simulink model "gantry_2025a"  (R2025a)
settings: Solver=ode45  StartTime=0.0  StopTime=t(end)  RelTol=1e-4  AbsTol=1e-8
undefined symbols (not defined in the file): cb1, cb2, cc1, cc2, ccy, cg1, cg2, cy, d, Jb, Jh, kb1, kb2, Lb, Lh, m1, m2, mb, mh, P, ts, X, Y, Z
libraries: sm_lib x14, nesl_utility x10, cstblocks x3
settings Model: Creator=cocuser  LastModifiedBy=cocuser
settings DataIOCC: ReturnWorkspaceOutputs=off

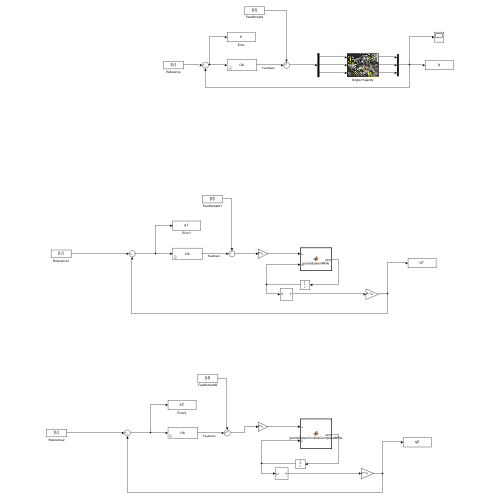
[thumbnail: Simulink's stored preview of the top-level diagram]
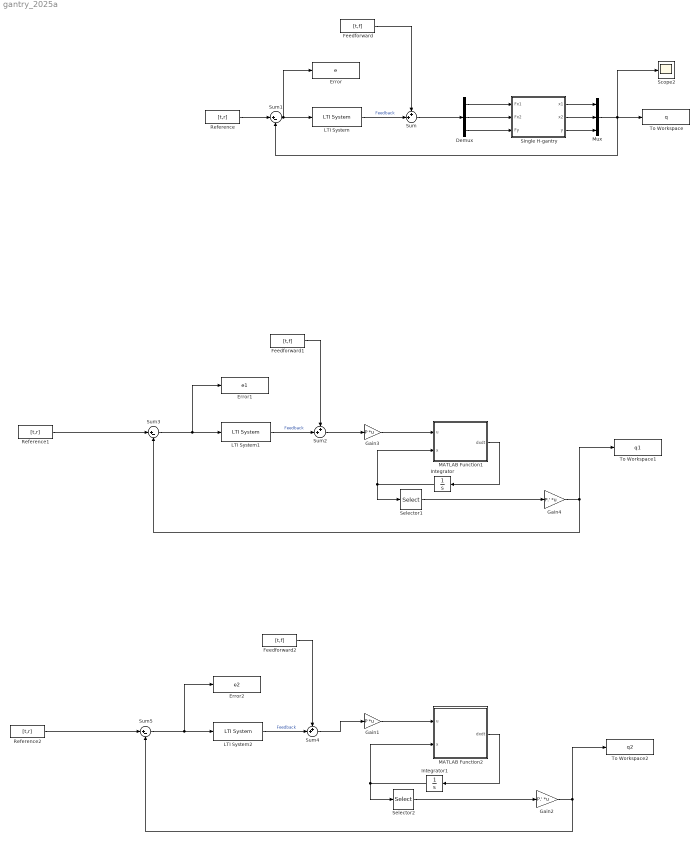
== system gantry_2025a ==
  Demux : Demux  Outputs=3
  Error : ToWorkspace  VariableName=e  SampleTime=ts
  Error1 : ToWorkspace  VariableName=e1  SampleTime=ts
  Error2 : ToWorkspace  VariableName=e2  SampleTime=ts
  Feedforward : FromWorkspace  VariableName=[t,f]  SampleTime=ts
  Feedforward1 : FromWorkspace  VariableName=[t,f]  SampleTime=ts
  Feedforward2 : FromWorkspace  VariableName=[t,f]  SampleTime=ts
  Gain1 : Gain  Gain=P  Multiplication=Matrix(K*u)
  Gain2 : Gain  Gain=P.'  Multiplication=Matrix(K*u)
  Gain3 : Gain  Gain=P  Multiplication=Matrix(K*u)
  Gain4 : Gain  Gain=P.'  Multiplication=Matrix(K*u)
  Integrator : Integrator  InitialCondition=[0;0;Y;0;0;0]
  Integrator1 : Integrator  InitialCondition=[0;0;Y;0;0;0]
  LTI System : cstblocks/LTI System  sys=Cfb  IC=[]  PadeOrder=0
  LTI System1 : cstblocks/LTI System  sys=Cfb  IC=[]  PadeOrder=0
  LTI System2 : cstblocks/LTI System  sys=Cfb  IC=[]  PadeOrder=0
  MATLAB Function1 : MATLAB Function  TreatAsAtomicUnit=on
  MATLAB Function2 : MATLAB Function  TreatAsAtomicUnit=on
  Mux : Mux  Inputs=3
  Reference : FromWorkspace  VariableName=[t,r]  SampleTime=ts
  Reference1 : FromWorkspace  VariableName=[t,r]  SampleTime=ts
  Reference2 : FromWorkspace  VariableName=[t,r]  SampleTime=ts
  Scope2 : Scope
      settings: ActiveDisplayYMinimum=-0.1624369949712226  ActiveDisplayYMaximum=0.46244043951976621  DataLoggingVariableName=ScopeData2
  Selector1 : Selector  InputPortWidth=6  IndexOptions=Index vector (dialog)  Indices=[1 2 3]  OutputSizes=1
  Selector2 : Selector  InputPortWidth=6  IndexOptions=Index vector (dialog)  Indices=[1 2 3]  OutputSizes=1
  Single H-gantry : Subsystem
      mask Display: image('h-gantry.png');
  Sum : Sum  Inputs=++|
  Sum1 : Sum  Inputs=|+-
  Sum2 : Sum  Inputs=++|
  Sum3 : Sum  Inputs=|+-
  Sum4 : Sum  Inputs=++|
  Sum5 : Sum  Inputs=|+-
  To Workspace : ToWorkspace  VariableName=q  SampleTime=ts
  To Workspace1 : ToWorkspace  VariableName=q1  SampleTime=ts
  To Workspace2 : ToWorkspace  VariableName=q2  SampleTime=ts
  wires:
  Single H-gantry/3(y) -> Mux/3
  Demux/1 -> Single H-gantry/1(Fx1)
  Demux/2 -> Single H-gantry/2(Fx2)
  Demux/3 -> Single H-gantry/3(Fy)
  Single H-gantry/1(x1) -> Mux/1
  Single H-gantry/2(x2) -> Mux/2
  Sum/1 -> Demux/1
  Feedforward/1 -> Sum/1
  Reference/1 -> Sum1/1
  Mux/1 -> Scope2/1, Sum1/2, To Workspace/1
  LTI System/1 -> Sum/2  "Feedback"
  Sum1/1 -> Error/1, LTI System/1
  LTI System1/1 -> Sum2/2  "Feedback"
  Feedforward1/1 -> Sum2/1
  Sum3/1 -> Error1/1, LTI System1/1
  Integrator/1 -> MATLAB Function1/2(x), Selector1/1
  Selector1/1 -> Gain4/1
  Sum2/1 -> Gain3/1
  Gain3/1 -> MATLAB Function1/1(u)
  Gain4/1 -> To Workspace1/1, Sum3/2
  MATLAB Function1/1(dxdt) -> Integrator/1
  Reference1/1 -> Sum3/1
  Sum4/1 -> Gain1/1
  Gain1/1 -> MATLAB Function2/1(u)
  LTI System2/1 -> Sum4/2  "Feedback"
  Gain2/1 -> To Workspace2/1, Sum5/2
  Reference2/1 -> Sum5/1
  Feedforward2/1 -> Sum4/1
  MATLAB Function2/1(dxdt) -> Integrator1/1
  Selector2/1 -> Gain2/1
  Integrator1/1 -> MATLAB Function2/2(x), Selector2/1
  Sum5/1 -> Error2/1, LTI System2/1

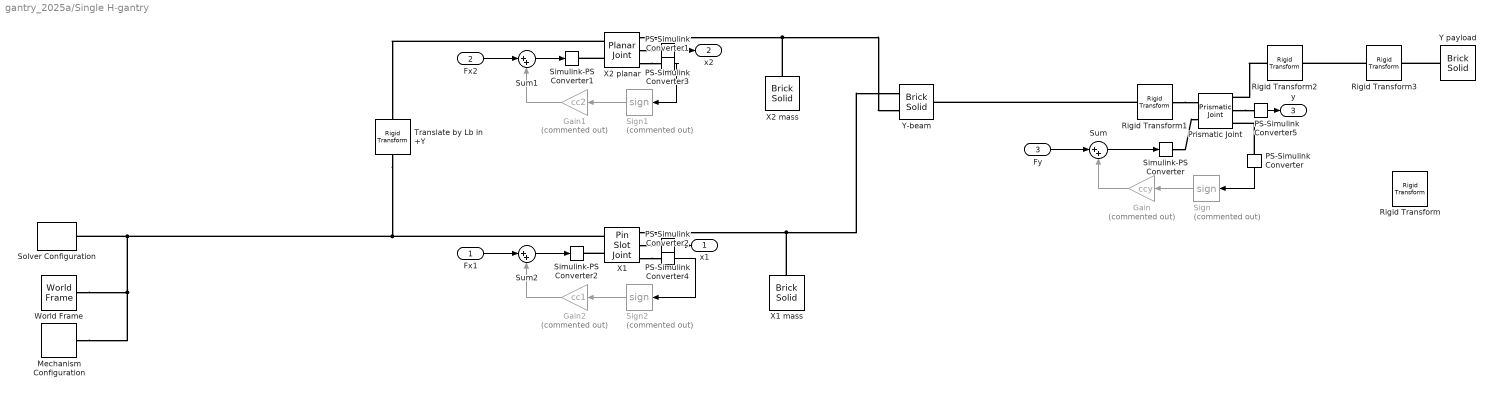
== system gantry_2025a/Single H-gantry ==
  Fx1 : Inport
  Fx2 : Inport  Port=2
  Fy : Inport  Port=3
  Gain : Gain  Commented=on  Gain=ccy
  Gain1 : Gain  Commented=on  Gain=cc2
  Gain2 : Gain  Commented=on  Gain=cc1
  Mechanism Configuration : sm_lib/Utilities/Mechanism Configuration  UniformGravity=Constant  GravityVector=[0 0 0]  GravityVectorUnits=m/s^2  LinearizationDelta=0.001  JointModeTransitionNonlinearIterations=2
  PS-Simulink Converter{,1..5} (6 alike) : nesl_utility/PS-Simulink Converter  PhysicalDomain=network_engine_domain  SubClassName=ps_output  LeftPortType=input  RightPortType=output  PseudoPeriodic=off  Frequencies=[]  VectorFormat=inherit  Unit=inherit  AffineConversion=off
  Prismatic Joint : sm_lib/Joints/Prismatic Joint  JointMode=Normal  CompositeWrenchDir=FollowerOnBase  CompositeWrenchFrame=BaseFrame  SenseConstraintForce=off  SenseConstraintTorque=off  SenseTotalForce=off  SenseTotalTorque=off  PositionTargetSpecify=on  PositionTargetPriority=High  PositionTargetValue=Y  PositionTargetValueUnits=m  VelocityTargetSpecify=off  VelocityTargetPriority=High  VelocityTargetValue=0  VelocityTargetValueUnits=m/s  EquilibriumPosition=0  EquilibriumPositionUnits=m  SpringStiffness=0  SpringStiffnessUnits=N/m  DampingCoefficient=cy  DampingCoefficientUnits=N/(m/s)  LowerLimitSpecify=off  LowerLimitBound=-1  LowerLimitBoundUnits=m  LowerLimitStiffness=1e6  LowerLimitStiffnessUnits=N/m  LowerLimitDamping=1e3  LowerLimitDampingUnits=N/(m/s)  LowerLimitTransitionRegionWidth=1e-4  LowerLimitTransitionRegionWidthUnits=m  UpperLimitSpecify=off  UpperLimitBound=1  UpperLimitBoundUnits=m  UpperLimitStiffness=1e6  UpperLimitStiffnessUnits=N/m  UpperLimitDamping=1e3  UpperLimitDampingUnits=N/(m/s)  UpperLimitTransitionRegionWidth=1e-4  UpperLimitTransitionRegionWidthUnits=m  TorqueActuationMode=InputTorque  MotionActuationMode=ComputedMotion  SensePosition=on  SenseVelocity=on  SenseAcceleration=off  SenseTorqueForce=off  SenseLowerLimitTorqueForce=off  SenseUpperLimitTorqueForce=off
  Rigid Transform : sm_lib/Frames and Transforms/Rigid Transform  RotationMethod=None  FollAlignAxisA=+X  BaseAlignAxisA=+Y  FollAlignAxisB=+Y  BaseAlignAxisB=+Z  RotationStandardAxis=+Z  RotationAngle=0  RotationAngleUnits=deg  RotationArbitraryAxis=[0 0 1]  RotationSequenceAxes=FollowerAxes  RotationSequence=XYX  RotationSequenceAngles=[0 0 0]  RotationSequenceAnglesUnits=deg  RotationMatrix=[1 0 0;0 1 0;0 0 1]  Quaternion=[1 0 0 0]  TranslationMethod=Cartesian  TranslationCartesianOffset=[-d 0 0]  TranslationCartesianOffsetUnits=m  TranslationStandardAxis=+Z  TranslationStandardOffset=0  TranslationStandardOffsetUnits=m  TranslationROffset=0  TranslationROffsetUnits=m  TranslationThetaOffset=0  TranslationThetaOffsetUnits=deg  TranslationZOffset=0  TranslationZOffsetUnits=m
  Rigid Transform1 : sm_lib/Frames and Transforms/Rigid Transform  RotationMethod=StandardAxis  FollAlignAxisA=+X  BaseAlignAxisA=+Y  FollAlignAxisB=+Y  BaseAlignAxisB=+Z  RotationStandardAxis=+X  RotationAngle=-90  RotationAngleUnits=deg  RotationArbitraryAxis=[0 0 1]  RotationSequenceAxes=FollowerAxes  RotationSequence=XYX  RotationSequenceAngles=[0 0 0]  RotationSequenceAnglesUnits=deg  RotationMatrix=[1 0 0;0 1 0;0 0 1]  Quaternion=[1 0 0 0]  TranslationMethod=None  TranslationCartesianOffset=[0 0 0]  TranslationCartesianOffsetUnits=m  TranslationStandardAxis=+Z  TranslationStandardOffset=0  TranslationStandardOffsetUnits=m  TranslationROffset=0  TranslationROffsetUnits=m  TranslationThetaOffset=0  TranslationThetaOffsetUnits=deg  TranslationZOffset=0  TranslationZOffsetUnits=m
  Rigid Transform2 : sm_lib/Frames and Transforms/Rigid Transform  RotationMethod=StandardAxis  FollAlignAxisA=+X  BaseAlignAxisA=+Y  FollAlignAxisB=+Y  BaseAlignAxisB=+Z  RotationStandardAxis=+X  RotationAngle=-90  RotationAngleUnits=deg  RotationArbitraryAxis=[0 0 1]  RotationSequenceAxes=FollowerAxes  RotationSequence=XYX  RotationSequenceAngles=[0 0 0]  RotationSequenceAnglesUnits=deg  RotationMatrix=[1 0 0;0 1 0;0 0 1]  Quaternion=[1 0 0 0]  TranslationMethod=None  TranslationCartesianOffset=[0 0 0]  TranslationCartesianOffsetUnits=m  TranslationStandardAxis=+Z  TranslationStandardOffset=0  TranslationStandardOffsetUnits=m  TranslationROffset=0  TranslationROffsetUnits=m  TranslationThetaOffset=0  TranslationThetaOffsetUnits=deg  TranslationZOffset=0  TranslationZOffsetUnits=m
  Rigid Transform3 : sm_lib/Frames and Transforms/Rigid Transform  RotationMethod=None  FollAlignAxisA=+X  BaseAlignAxisA=+Y  FollAlignAxisB=+Y  BaseAlignAxisB=+Z  RotationStandardAxis=+Z  RotationAngle=0  RotationAngleUnits=deg  RotationArbitraryAxis=[0 0 1]  RotationSequenceAxes=FollowerAxes  RotationSequence=XYX  RotationSequenceAngles=[0 0 0]  RotationSequenceAnglesUnits=deg  RotationMatrix=[1 0 0;0 1 0;0 0 1]  Quaternion=[1 0 0 0]  TranslationMethod=Cartesian  TranslationCartesianOffset=[-d 0 0]  TranslationCartesianOffsetUnits=m  TranslationStandardAxis=+Z  TranslationStandardOffset=0  TranslationStandardOffsetUnits=m  TranslationROffset=0  TranslationROffsetUnits=m  TranslationThetaOffset=0  TranslationThetaOffsetUnits=deg  TranslationZOffset=0  TranslationZOffsetUnits=m
  Sign : Signum  Commented=on
  Sign1 : Signum  Commented=on
  Sign2 : Signum  Commented=on
  Simulink-PS Converter : nesl_utility/Simulink-PS Converter  PhysicalDomain=network_engine_domain  SubClassName=ps_input  LeftPortType=input  RightPortType=output  PseudoPeriodic=off  Frequencies=[]  NoiseDistribution=none  NoiseParameters=[]  Unit=1  AffineConversion=off  FilteringAndDerivatives=provide  SimscapeFilterOrder=1  InputFilterTimeConstant=0.001  UdotUserProvided=0
  Simulink-PS Converter1 : nesl_utility/Simulink-PS Converter  PhysicalDomain=network_engine_domain  SubClassName=ps_input  LeftPortType=input  RightPortType=output  PseudoPeriodic=off  Frequencies=[]  NoiseDistribution=none  NoiseParameters=[]  Unit=1  AffineConversion=off  FilteringAndDerivatives=provide  SimscapeFilterOrder=1  InputFilterTimeConstant=0.001  UdotUserProvided=0
  Simulink-PS Converter2 : nesl_utility/Simulink-PS Converter  PhysicalDomain=network_engine_domain  SubClassName=ps_input  LeftPortType=input  RightPortType=output  PseudoPeriodic=off  Frequencies=[]  NoiseDistribution=none  NoiseParameters=[]  Unit=1  AffineConversion=off  FilteringAndDerivatives=provide  SimscapeFilterOrder=1  InputFilterTimeConstant=0.001  UdotUserProvided=0
  Solver Configuration : nesl_utility/Solver Configuration  PhysicalDomain=network_engine_domain  SubClassName=solver  LeftPortType=input  RightPortType=generic  Tones=[]  Harmonics=[]  SimulateNoise=off  Profile=off  UseLocalSampling=off  EnableSwitchedLinearOptims=on  FrequencyDomain=off  UseCCode=off  RelTol=0.001  AbsTol=0.001  MinStep=1e-09  ToWorkspace=off  RevertToSquareIcSolve=off  NumHomotopyIterations=100  PhasorMode=off  PhasorModeNumHarmonics=1  ConsistencySolver=NEWTON_XTOL_AFTER_FTOL  IndexReductionMethod=DerivativeReplacement  DoDC=off  ResidualTolerance=1e-09  ConsistencyTolSource=GLOBAL  ConsistencyAbsTol=0.001  ConsistencyRelTol=0.001  ConsistencyTolFactor=1e-3  UseLocalSolver=off  LocalSolverChoice=NE_BACKWARD_EULER_ADVANCER  ResolveIndetEquations=on  FunctionEvalNumThread=1  LocalSolverSampleTime=0.001  DoFixedCost=off  MaxNonlinIter=3  MaxModeIter=2  ComputeImpulses=off  ImpulseIterations=2  LinearAlgebra=auto  LinearAlgebraNumThread=0  EquationFormulation=NE_TIME_EF  DelaysMemoryBudget=1024  AutomaticFiltering=on  FilteringTimeConstant=0.001  PartitionStorageMethod=AS_NEEDED  PartitionMemoryBudget=1024  PartitionMethod=ROBUST  MultibodyUseLocalSolver=off  MultibodyLocalSolverChoice=ODE1  MultibodyLocalSolverSampleTime=0.001
  Sum : Sum  Inputs=|++
  Sum1 : Sum  Inputs=|++
  Sum2 : Sum  Inputs=|++
  Translate by Lb in +Y : sm_lib/Frames and Transforms/Rigid Transform  RotationMethod=None  FollAlignAxisA=+X  BaseAlignAxisA=+Y  FollAlignAxisB=+Y  BaseAlignAxisB=+Z  RotationStandardAxis=+Z  RotationAngle=0  RotationAngleUnits=deg  RotationArbitraryAxis=[0 0 1]  RotationSequenceAxes=FollowerAxes  RotationSequence=XYX  RotationSequenceAngles=[0 0 0]  RotationSequenceAnglesUnits=deg  RotationMatrix=[1 0 0;0 1 0;0 0 1]  Quaternion=[1 0 0 0]  TranslationMethod=Cartesian  TranslationCartesianOffset=[0 Lb 0]  TranslationCartesianOffsetUnits=m  TranslationStandardAxis=+Z  TranslationStandardOffset=0  TranslationStandardOffsetUnits=m  TranslationROffset=0  TranslationROffsetUnits=m  TranslationThetaOffset=0  TranslationThetaOffsetUnits=deg  TranslationZOffset=0  TranslationZOffsetUnits=m
  World Frame : sm_lib/Frames and Transforms/World Frame
  X1 : sm_lib/Joints/Pin Slot Joint  JointMode=Normal  CompositeWrenchDir=FollowerOnBase  CompositeWrenchFrame=BaseFrame  SenseConstraintForce=off  SenseConstraintTorque=off  SenseTotalForce=off  SenseTotalTorque=off  PxPositionTargetSpecify=off  PxPositionTargetPriority=High  PxPositionTargetValue=0  PxPositionTargetValueUnits=m  PxVelocityTargetSpecify=off  PxVelocityTargetPriority=High  PxVelocityTargetValue=0  PxVelocityTargetValueUnits=m/s  PxEquilibriumPosition=0  PxEquilibriumPositionUnits=m  PxSpringStiffness=0  PxSpringStiffnessUnits=N/m  PxDampingCoefficient=cg1  PxDampingCoefficientUnits=N/(m/s)  PxLowerLimitSpecify=off  PxLowerLimitBound=-1  PxLowerLimitBoundUnits=m  PxLowerLimitStiffness=1e6  PxLowerLimitStiffnessUnits=N/m  PxLowerLimitDamping=1e3  PxLowerLimitDampingUnits=N/(m/s)  PxLowerLimitTransitionRegionWidth=1e-4  PxLowerLimitTransitionRegionWidthUnits=m  PxUpperLimitSpecify=off  PxUpperLimitBound=1  PxUpperLimitBoundUnits=m  PxUpperLimitStiffness=1e6  PxUpperLimitStiffnessUnits=N/m  PxUpperLimitDamping=1e3  PxUpperLimitDampingUnits=N/(m/s)  PxUpperLimitTransitionRegionWidth=1e-4  PxUpperLimitTransitionRegionWidthUnits=m  PxTorqueActuationMode=InputTorque  PxMotionActuationMode=ComputedMotion  PxSensePosition=on  PxSenseVelocity=on  PxSenseAcceleration=off  PxSenseTorqueForce=off  PxSenseLowerLimitTorqueForce=off  PxSenseUpperLimitTorqueForce=off  RzPositionTargetSpecify=off  RzPositionTargetPriority=High  RzPositionTargetValue=0  RzPositionTargetValueUnits=deg  RzVelocityTargetSpecify=off  RzVelocityTargetPriority=High  RzVelocityTargetValue=0  RzVelocityTargetValueUnits=deg/s  RzEquilibriumPosition=0  RzEquilibriumPositionUnits=rad  RzSpringStiffness=kb1  RzSpringStiffnessUnits=N*m/rad  RzDampingCoefficient=cb1  RzDampingCoefficientUnits=N*m*s/rad  RzLowerLimitSpecify=off  RzLowerLimitBound=-90  RzLowerLimitBoundUnits=deg  RzLowerLimitStiffness=1e4  RzLowerLimitStiffnessUnits=N*m/deg  RzLowerLimitDamping=10  RzLowerLimitDampingUnits=N*m/(deg/s)  RzLowerLimitTransitionRegionWidth=0.1  RzLowerLimitTransitionRegionWidthUnits=deg  RzUpperLimitSpecify=off  RzUpperLimitBound=90  RzUpperLimitBoundUnits=deg  RzUpperLimitStiffness=1e4  RzUpperLimitStiffnessUnits=N*m/deg  RzUpperLimitDamping=10  RzUpperLimitDampingUnits=N*m/(deg/s)  RzUpperLimitTransitionRegionWidth=0.1  RzUpperLimitTransitionRegionWidthUnits=deg  RzTorqueActuationMode=NoTorque  RzMotionActuationMode=ComputedMotion  RzSensePosition=off  RzSenseVelocity=off  RzSenseAcceleration=off  RzSenseTorqueForce=off  RzSenseLowerLimitTorqueForce=off  RzSenseUpperLimitTorqueForce=off
  X1 mass : sm_lib/Body Elements/Brick Solid  BrickDimensions=1e-1*[1 1 1]  BrickDimensionsUnits=m  ExportEntireGeometry=off  InertiaType=PointMass  BasedOnType=Mass  Density=1000  DensityUnits=kg/m^3  Mass=m1  MassUnits=kg  CenterOfMass=[0 0 0]  CenterOfMassUnits=m  MomentsOfInertia=[1 1 1]  MomentsOfInertiaUnits=kg*m^2  ProductsOfInertia=[0 0 0]  ProductsOfInertiaUnits=kg*m^2  GraphicType=FromGeometry  MarkerShape=Sphere  MarkerSize=10  GraphicVisPropType=SimpleVisualProperties  GraphicDiffuseColor=[0.8157 0 0]  GraphicOpacity=1  GraphicSpecularColor=[0.5 0.5 0.5 1.0]  GraphicAmbientColor=[0.15 0.15 0.15 1.0]  GraphicEmissiveColor=[0.0 0.0 0.0 1.0]  GraphicShininess=75  DoExposeReferenceFrame=on  SerializedFrames=<Frames/>
  X2 mass : sm_lib/Body Elements/Brick Solid  BrickDimensions=1e-1*[1 1 1]  BrickDimensionsUnits=m  ExportEntireGeometry=off  InertiaType=PointMass  BasedOnType=Mass  Density=1000  DensityUnits=kg/m^3  Mass=m2  MassUnits=kg  CenterOfMass=[0 0 0]  CenterOfMassUnits=m  MomentsOfInertia=[1 1 1]  MomentsOfInertiaUnits=kg*m^2  ProductsOfInertia=[0 0 0]  ProductsOfInertiaUnits=kg*m^2  GraphicType=FromGeometry  MarkerShape=Sphere  MarkerSize=10  GraphicVisPropType=SimpleVisualProperties  GraphicDiffuseColor=[0.8157 0 0]  GraphicOpacity=1  GraphicSpecularColor=[0.5 0.5 0.5 1.0]  GraphicAmbientColor=[0.15 0.15 0.15 1.0]  GraphicEmissiveColor=[0.0 0.0 0.0 1.0]  GraphicShininess=75  DoExposeReferenceFrame=on  SerializedFrames=<Frames/>
  X2 planar : sm_lib/Joints/Planar Joint  JointMode=Normal  CompositeWrenchDir=FollowerOnBase  CompositeWrenchFrame=BaseFrame  SenseConstraintForce=off  SenseConstraintTorque=off  SenseTotalForce=off  SenseTotalTorque=off  PxPositionTargetSpecify=off  PxPositionTargetPriority=High  PxPositionTargetValue=0  PxPositionTargetValueUnits=m  PxVelocityTargetSpecify=off  PxVelocityTargetPriority=High  PxVelocityTargetValue=0  PxVelocityTargetValueUnits=m/s  PxEquilibriumPosition=0  PxEquilibriumPositionUnits=m  PxSpringStiffness=0  PxSpringStiffnessUnits=N/m  PxDampingCoefficient=cg2  PxDampingCoefficientUnits=N/(m/s)  PxLowerLimitSpecify=off  PxLowerLimitBound=-1  PxLowerLimitBoundUnits=m  PxLowerLimitStiffness=1e6  PxLowerLimitStiffnessUnits=N/m  PxLowerLimitDamping=1e3  PxLowerLimitDampingUnits=N/(m/s)  PxLowerLimitTransitionRegionWidth=1e-4  PxLowerLimitTransitionRegionWidthUnits=m  PxUpperLimitSpecify=off  PxUpperLimitBound=1  PxUpperLimitBoundUnits=m  PxUpperLimitStiffness=1e6  PxUpperLimitStiffnessUnits=N/m  PxUpperLimitDamping=1e3  PxUpperLimitDampingUnits=N/(m/s)  PxUpperLimitTransitionRegionWidth=1e-4  PxUpperLimitTransitionRegionWidthUnits=m  PxTorqueActuationMode=InputTorque  PxMotionActuationMode=ComputedMotion  PxSensePosition=on  PxSenseVelocity=on  PxSenseAcceleration=off  PxSenseTorqueForce=off  PxSenseLowerLimitTorqueForce=off  PxSenseUpperLimitTorqueForce=off  PyPositionTargetSpecify=off  PyPositionTargetPriority=High  PyPositionTargetValue=0  PyPositionTargetValueUnits=m  PyVelocityTargetSpecify=off  PyVelocityTargetPriority=High  PyVelocityTargetValue=0  PyVelocityTargetValueUnits=m/s  PyEquilibriumPosition=0  PyEquilibriumPositionUnits=m  PySpringStiffness=0  PySpringStiffnessUnits=N/m  PyDampingCoefficient=0  PyDampingCoefficientUnits=N/(m/s)  PyLowerLimitSpecify=off  PyLowerLimitBound=-1  PyLowerLimitBoundUnits=m  PyLowerLimitStiffness=1e6  PyLowerLimitStiffnessUnits=N/m  PyLowerLimitDamping=1e3  PyLowerLimitDampingUnits=N/(m/s)  PyLowerLimitTransitionRegionWidth=1e-4  PyLowerLimitTransitionRegionWidthUnits=m  PyUpperLimitSpecify=off  PyUpperLimitBound=1  PyUpperLimitBoundUnits=m  PyUpperLimitStiffness=1e6  PyUpperLimitStiffnessUnits=N/m  PyUpperLimitDamping=1e3  PyUpperLimitDampingUnits=N/(m/s)  PyUpperLimitTransitionRegionWidth=1e-4  PyUpperLimitTransitionRegionWidthUnits=m  PyTorqueActuationMode=NoTorque  PyMotionActuationMode=ComputedMotion  PySensePosition=off  PySenseVelocity=off  PySenseAcceleration=off  PySenseTorqueForce=off  PySenseLowerLimitTorqueForce=off  PySenseUpperLimitTorqueForce=off  RzPositionTargetSpecify=off  RzPositionTargetPriority=High  RzPositionTargetValue=0  RzPositionTargetValueUnits=deg  RzVelocityTargetSpecify=off  RzVelocityTargetPriority=High  RzVelocityTargetValue=0  RzVelocityTargetValueUnits=deg/s  RzEquilibriumPosition=0  RzEquilibriumPositionUnits=rad  RzSpringStiffness=kb2  RzSpringStiffnessUnits=N*m/rad  RzDampingCoefficient=cb2  RzDampingCoefficientUnits=N*m*s/rad  RzLowerLimitSpecify=off  RzLowerLimitBound=-90  RzLowerLimitBoundUnits=deg  RzLowerLimitStiffness=1e4  RzLowerLimitStiffnessUnits=N*m/deg  RzLowerLimitDamping=10  RzLowerLimitDampingUnits=N*m/(deg/s)  RzLowerLimitTransitionRegionWidth=0.1  RzLowerLimitTransitionRegionWidthUnits=deg  RzUpperLimitSpecify=off  RzUpperLimitBound=90  RzUpperLimitBoundUnits=deg  RzUpperLimitStiffness=1e4  RzUpperLimitStiffnessUnits=N*m/deg  RzUpperLimitDamping=10  RzUpperLimitDampingUnits=N*m/(deg/s)  RzUpperLimitTransitionRegionWidth=0.1  RzUpperLimitTransitionRegionWidthUnits=deg  RzTorqueActuationMode=NoTorque  RzMotionActuationMode=ComputedMotion  RzSensePosition=off  RzSenseVelocity=off  RzSenseAcceleration=off  RzSenseTorqueForce=off  RzSenseLowerLimitTorqueForce=off  RzSenseUpperLimitTorqueForce=off
  Y payload : sm_lib/Body Elements/Brick Solid  BrickDimensions=[Lh/2 Lh Lh/2]  BrickDimensionsUnits=m  ExportEntireGeometry=off  InertiaType=Custom  BasedOnType=Mass  Density=1000  DensityUnits=kg/m^3  Mass=mh  MassUnits=kg  CenterOfMass=[0 0 0]  CenterOfMassUnits=m  MomentsOfInertia=[1 1 Jh]  MomentsOfInertiaUnits=kg*m^2  ProductsOfInertia=[0 0 0]  ProductsOfInertiaUnits=kg*m^2  GraphicType=FromGeometry  MarkerShape=Sphere  MarkerSize=10  GraphicVisPropType=SimpleVisualProperties  GraphicDiffuseColor=[0 0.6667 1]  GraphicOpacity=1  GraphicSpecularColor=[0.5 0.5 0.5 1.0]  GraphicAmbientColor=[0.15 0.15 0.15 1.0]  GraphicEmissiveColor=[0.0 0.0 0.0 1.0]  GraphicShininess=75  DoExposeReferenceFrame=on  SerializedFrames=<Frames/>
  Y-beam : sm_lib/Body Elements/Brick Solid  BrickDimensions=[Lh/2 Lb Lh/2]  BrickDimensionsUnits=m  ExportEntireGeometry=off  InertiaType=Custom  BasedOnType=Density  Density=1000  DensityUnits=kg/m^3  Mass=mb  MassUnits=kg  CenterOfMass=[0 0 0]  CenterOfMassUnits=m  MomentsOfInertia=[1 1 Jb]  MomentsOfInertiaUnits=kg*m^2  ProductsOfInertia=[0 0 0]  ProductsOfInertiaUnits=kg*m^2  GraphicType=FromGeometry  MarkerShape=Sphere  MarkerSize=10  GraphicVisPropType=SimpleVisualProperties  GraphicDiffuseColor=[0 0.8627 0]  GraphicOpacity=1  GraphicSpecularColor=[0.5 0.5 0.5 1.0]  GraphicAmbientColor=[0.15 0.15 0.15 1.0]  GraphicEmissiveColor=[0.0 0.0 0.0 1.0]  GraphicShininess=75  DoExposeReferenceFrame=on  SerializedFrames=|
      | <Frames>
      | 
      |   <Frame>
      |     <Id>Frame1</Id>
      |     <Value>
      |       <Name>X1</Name>
      |       <Origin>
      |         <Source>GeometricFeature</Source>
      |         <FeatureName>-y surface</FeatureName>
      |       </Origin>
      |       <PrimaryAxis>
      |         <DefinedDirection>+Z</DefinedDirection>
      |         <Source>ReferenceFrame</Source>
      |         <SourceDirection>+Z</SourceDirection>
      |         <FeatureName></FeatureName>
      |       </PrimaryAxis>
      |       <SecondaryAxis>
      |         <DefinedDirection>+X</DefinedDirection>
      |         <Source>ReferenceFrame</Source>
      |         <SourceDirection>+X</SourceDirection>
      |         <FeatureName></FeatureName>
      |       </SecondaryAxis>
      |     </Value>
      |   </Frame>
      | 
      |   <Frame>
      |     <Id>Frame2</Id>
      |     <Value>
      |       <Name>X2</Name>
      |       <Origin>
      |         <Source>GeometricFeature</Source>
      |         <FeatureName>+y surface</FeatureName>
      |       </Origin>
      |       <PrimaryAxis>
      |         <DefinedDirection>+Z</DefinedDirection>
      |         <Source>ReferenceFrame</Source>
      |         <SourceDirection>+Z</SourceDirection>
      |         <FeatureName></FeatureName>
      |       </PrimaryAxis>
      |       <SecondaryAxis>
      |         <DefinedDirection>+X</DefinedDirection>
      |         <Source>ReferenceFrame</Source>
      |         <SourceDirection>+X</SourceDirection>
      |         <FeatureName></FeatureName>
      |       </SecondaryAxis>
      |     </Value>
      |   </Frame>
      | 
      | </Frames>
  x1 : Outport
  x2 : Outport  Port=2
  y : Outport  Port=3
  wires:
  PS-Simulink Converter2/1 -> Sign2/1
  Gain2/1 -> Sum2/2
  Sign2/1 -> Gain2/1
  Sign1/1 -> Gain1/1
  Fy/1 -> Sum/1
  Gain/1 -> Sum/2
  PS-Simulink Converter1/1 -> Sign1/1
  Sum2/1 -> Simulink-PS Converter2/1
  Gain1/1 -> Sum1/2
  Sum1/1 -> Simulink-PS Converter1/1
  Sign/1 -> Gain/1
  Fx1/1 -> Sum2/1
  Sum/1 -> Simulink-PS Converter/1
  PS-Simulink Converter/1 -> Sign/1
  Fx2/1 -> Sum1/1
  PS-Simulink Converter3/1 -> x2/1
  PS-Simulink Converter4/1 -> x1/1
  PS-Simulink Converter5/1 -> y/1
  connections:
  Simulink-PS Converter/RConn1 -- Prismatic Joint/LConn2
  X2 planar/LConn2 -- Simulink-PS Converter1/RConn1
  Y payload/RConn1 -- Rigid Transform3/RConn1
  X2 planar/RConn3 -- PS-Simulink Converter1/LConn1
  X2 planar/LConn1 -- Translate by Lb in +Y/RConn1
  X2 mass/RConn1 -- X2 planar/RConn1 -- Y-beam/LConn2
  Rigid Transform2/LConn1 -- Prismatic Joint/RConn1
  X1 mass/RConn1 -- X1/RConn1 -- Y-beam/LConn1
  X1/RConn3 -- PS-Simulink Converter2/LConn1
  Rigid Transform1/LConn1 -- Y-beam/RConn1
  Rigid Transform1/RConn1 -- Prismatic Joint/LConn1
  PS-Simulink Converter/LConn1 -- Prismatic Joint/RConn3
  X1/LConn2 -- Simulink-PS Converter2/RConn1
  X2 planar/RConn2 -- PS-Simulink Converter3/LConn1
  X1/RConn2 -- PS-Simulink Converter4/LConn1
  Prismatic Joint/RConn2 -- PS-Simulink Converter5/LConn1
  Translate by Lb in +Y/LConn1 -- X1/LConn1 -- Mechanism Configuration/RConn1 -- World Frame/RConn1 -- Solver Configuration/RConn1
  Rigid Transform3/LConn1 -- Rigid Transform2/RConn1

== matlab function gantry_2025a/MATLAB Function1 ==
  data: dxdt output; u input; x input; m1 parameter; m2 parameter; mb parameter; mh parameter; Jb parameter; Jh parameter; d parameter; Lb parameter; kb1 parameter; kb2 parameter; cg1 parameter; cg2 parameter; cb1 parameter; cb2 parameter; cy parameter
function dxdt = gantrySystemMFile(u,x,m1,m2,mb,mh,Jb,Jh,d,Lb,kb1,kb2,cg1,cg2,cb1,cb2,cy)
dxdt = gantrySystem(u,x,m1,m2,mb,mh,Lb,Jb,Jh,d,cg1,cg2,cb1,cb2,cy,kb1,kb2); 
end

== matlab function gantry_2025a/MATLAB Function2 ==
  data: dxdt output; u input; x input; m1 parameter; m2 parameter; mb parameter; mh parameter; Jb parameter; Jh parameter; d parameter; Lb parameter; kb1 parameter; kb2 parameter; cg1 parameter; cg2 parameter; cb1 parameter; cb2 parameter; cy parameter
function dxdt = gantrySystemCoriolisCentripetalMFile(u,x,m1,m2,mb,mh,Jb,Jh,d,Lb,kb1,kb2,cg1,cg2,cb1,cb2,cy)
dxdt = gantrySystemCoriolisCentripetal(u,x,m1,m2,mb,mh,Jb,Jh,d,Lb,kb1,kb2,cg1,cg2,cb1,cb2,cy); 
end
